simulink model "hw1_model"  (R2024b)
settings: Solver=ode14x  StartTime=0.0  StopTime=44.0  FixedStep=0.001  RelTol=1e-3
undefined symbols (not defined in the file): Cd, Crr, Cxf, Cxr, Cyf, Cyr, F_max_x, F_max_y, Frontal_area, g, J, Jt, lf, lr, m, R, ro, slope
settings Model: Creator=Atakan  LastModifiedBy=Atakan

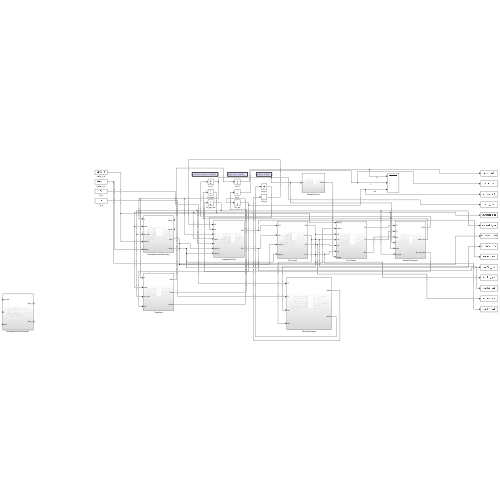
[thumbnail: Simulink's stored preview of the top-level diagram]
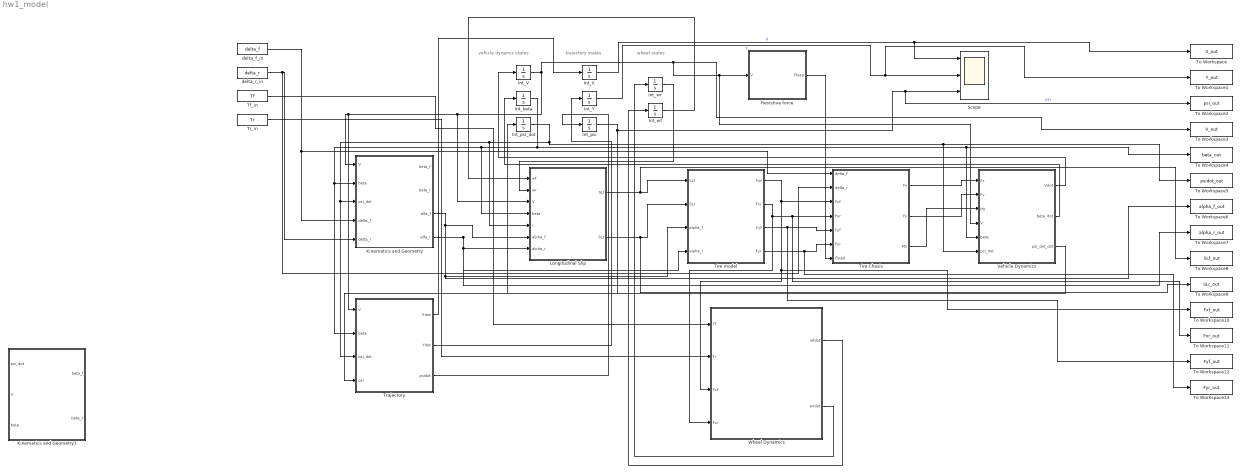
== system hw1_model ==
  note: wheel states
  note: trajectory states
  note: vehicle dynamic states
  Int_V : Integrator
  Int_X : Integrator
  Int_Y : Integrator
  Int_beta : Integrator
  Int_psi : Integrator
  Int_psi_dot : Integrator
  Int_wf : Integrator
  Int_wr : Integrator
  Kinematics and Geometry : Subsystem
  Kinematics and Geometry1 : Subsystem
  Longitudinal Slip : Subsystem
  Resistive force : Subsystem
  Scope : Scope  NumInputPorts=3
  Tf_in : FromWorkspace  VariableName=Tf
  "Tire Chasis " : Subsystem
  Tire model : Subsystem
  To Workspace : ToWorkspace  VariableName=X_out  SaveFormat=Structure With Time  SampleTime=-1
  To Workspace1 : ToWorkspace  VariableName=Y_out  SaveFormat=Structure With Time  SampleTime=-1
  To Workspace10 : ToWorkspace  VariableName=Fxf_out  SaveFormat=Structure With Time  SampleTime=-1
  To Workspace11 : ToWorkspace  VariableName=Fxr_out  SaveFormat=Structure With Time  SampleTime=-1
  To Workspace12 : ToWorkspace  VariableName=Fyf_out  SaveFormat=Structure With Time  SampleTime=-1
  To Workspace13 : ToWorkspace  VariableName=Fyr_out  SaveFormat=Structure With Time  SampleTime=-1
  To Workspace2 : ToWorkspace  VariableName=psi_out  SaveFormat=Structure With Time  SampleTime=-1
  To Workspace3 : ToWorkspace  VariableName=V_out  SaveFormat=Structure With Time  SampleTime=-1
  To Workspace4 : ToWorkspace  VariableName=beta_out  SaveFormat=Structure With Time  SampleTime=-1
  To Workspace5 : ToWorkspace  VariableName=psidot_out  SaveFormat=Structure With Time  SampleTime=-1
  To Workspace6 : ToWorkspace  VariableName=alpha_f_out  SaveFormat=Structure With Time  SampleTime=-1
  To Workspace7 : ToWorkspace  VariableName=alpha_r_out  SaveFormat=Structure With Time  SampleTime=-1
  To Workspace8 : ToWorkspace  VariableName=SLf_out  SaveFormat=Structure With Time  SampleTime=-1
  To Workspace9 : ToWorkspace  VariableName=SLr_out  SaveFormat=Structure With Time  SampleTime=-1
  Tr_in : FromWorkspace  VariableName=Tr
  Trajectory : Subsystem
  Vehicle Dynamics : Subsystem
  Wheel Dynamics : Subsystem
  delta_f_in : FromWorkspace  VariableName=delta_f
  delta_r_in : FromWorkspace  VariableName=delta_r
  wires:
  Int_V/1 -> To Workspace3/1, Vehicle Dynamics/4(V), Resistive force/1(V), Trajectory/1(V), Kinematics and Geometry/1(V), Longitudinal Slip/3(V)
  Int_beta/1 -> To Workspace4/1, Vehicle Dynamics/5(beta), Longitudinal Slip/4(beta), Trajectory/2(beta), Kinematics and Geometry/2(beta)
  Int_psi_dot/1 -> To Workspace5/1, Vehicle Dynamics/6(psi_dot), Longitudinal Slip/5(r), Trajectory/3(psi_dot), Kinematics and Geometry/3(psi_dot)
  delta_f_in/1 -> "Tire Chasis "/1(delta_f), Kinematics and Geometry/4(delta_f)
  delta_r_in/1 -> "Tire Chasis "/2(delta_r), Kinematics and Geometry/5(delta_r)
  Int_wf/1 -> Longitudinal Slip/1(wf)
  Int_wr/1 -> Longitudinal Slip/2(wr)
  Longitudinal Slip/1(SLf) -> To Workspace8/1, Tire model/1(SLf)
  Longitudinal Slip/2(SLr) -> To Workspace9/1, Tire model/2(SLr)
  Kinematics and Geometry/3(alfa_f) -> Longitudinal Slip/6(alpha_f), To Workspace6/1, Tire model/3(alpha_f)
  Kinematics and Geometry/4(alfa_r) -> To Workspace7/1, Longitudinal Slip/7(alpha_r), Tire model/4(alpha_r)
  Tire model/1(Fxf) -> To Workspace10/1, Wheel Dynamics/3(Fxf), "Tire Chasis "/3(Fxf)
  Tire model/2(Fxr) -> Wheel Dynamics/4(Fxr), To Workspace11/1, "Tire Chasis "/4(Fxr)
  Tire model/3(Fyf) -> To Workspace12/1, "Tire Chasis "/5(Fyf)
  Tire model/4(Fyr) -> To Workspace13/1, "Tire Chasis "/6(Fyr)
  Resistive force/1(Fload) -> "Tire Chasis "/7(Fload)
  "Tire Chasis "/1(Fx) -> Vehicle Dynamics/1(Fx)
  "Tire Chasis "/2(Fy) -> Vehicle Dynamics/2(Fy)
  "Tire Chasis "/3(Mz) -> Vehicle Dynamics/3(Mz)
  Vehicle Dynamics/1(Vdot) -> Int_V/1
  Vehicle Dynamics/2(beta_dot) -> Int_beta/1
  Vehicle Dynamics/3(psi_dot_dot) -> Int_psi_dot/1
  Int_psi/1 -> To Workspace2/1, Scope/3, Trajectory/4(psi)  "psi"
  Trajectory/1(Xdot) -> Int_X/1
  Trajectory/2(Ydot) -> Int_Y/1
  Trajectory/3(psidot) -> Int_psi/1
  Tf_in/1 -> Wheel Dynamics/1(Tf)
  Tr_in/1 -> Wheel Dynamics/2(Tr)
  Wheel Dynamics/1(wfdot) -> Int_wf/1
  Wheel Dynamics/2(wrdot) -> Int_wr/1
  Int_X/1 -> To Workspace/1, Scope/1  "X"
  Int_Y/1 -> To Workspace1/1, Scope/2  "Y"

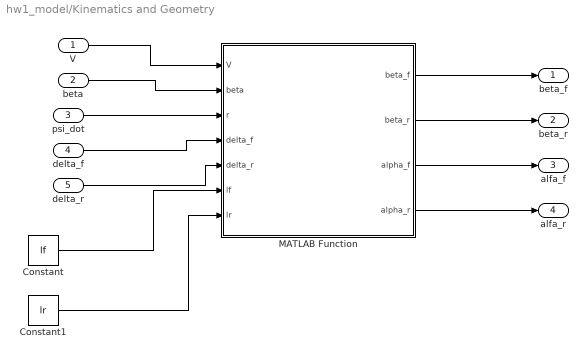
== system hw1_model/Kinematics and Geometry ==
  V : Inport
  beta : Inport  Port=2
  psi_dot : Inport  Port=3
  delta_f : Inport  Port=4
  delta_r : Inport  Port=5
  Constant : Constant  Value=lf
  Constant1 : Constant  Value=lr
  MATLAB Function : MATLAB Function  TreatAsAtomicUnit=on
  beta_f : Outport
  beta_r : Outport  Port=2
  alfa_f : Outport  Port=3
  alfa_r : Outport  Port=4
  wires:
  V/1 -> MATLAB Function/1(V)
  beta/1 -> MATLAB Function/2(beta)
  psi_dot/1 -> MATLAB Function/3(r)
  delta_f/1 -> MATLAB Function/4(delta_f)
  delta_r/1 -> MATLAB Function/5(delta_r)
  Constant/1 -> MATLAB Function/6(lf)
  Constant1/1 -> MATLAB Function/7(lr)
  MATLAB Function/1(beta_f) -> beta_f/1
  MATLAB Function/2(beta_r) -> beta_r/1
  MATLAB Function/3(alpha_f) -> alfa_f/1
  MATLAB Function/4(alpha_r) -> alfa_r/1

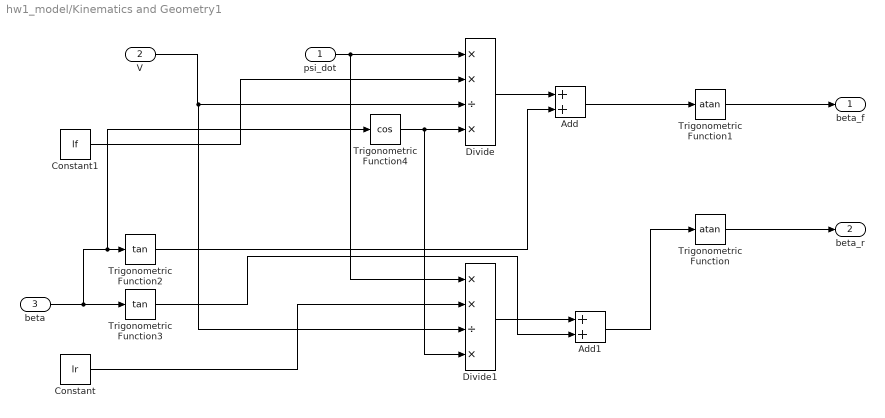
== system hw1_model/Kinematics and Geometry1 ==
  psi_dot : Inport
  V : Inport  Port=2
  beta : Inport  Port=3
  Add : Sum
  Add1 : Sum
  Constant : Constant  Value=lr
  Constant1 : Constant  Value=lf
  Divide : Product  Inputs=**/*
  Divide1 : Product  Inputs=**/*
  Trigonometric Function : Trigonometry  Operator=atan
  Trigonometric Function1 : Trigonometry  Operator=atan
  Trigonometric Function2 : Trigonometry  Operator=tan
  Trigonometric Function3 : Trigonometry  Operator=tan
  Trigonometric Function4 : Trigonometry  Operator=cos
  beta_f : Outport
  beta_r : Outport  Port=2
  wires:
  Trigonometric Function1/1 -> beta_f/1
  Trigonometric Function/1 -> beta_r/1
  beta/1 -> Trigonometric Function4/1, Trigonometric Function2/1, Trigonometric Function3/1
  psi_dot/1 -> Divide1/1, Divide/1
  Constant1/1 -> Divide/2
  V/1 -> Divide1/3, Divide/3
  Trigonometric Function4/1 -> Divide1/4, Divide/4
  Divide/1 -> Add/1
  Trigonometric Function2/1 -> Add/2
  Add/1 -> Trigonometric Function1/1
  Constant/1 -> Divide1/2
  Divide1/1 -> Add1/1
  Trigonometric Function3/1 -> Add1/2
  Add1/1 -> Trigonometric Function/1

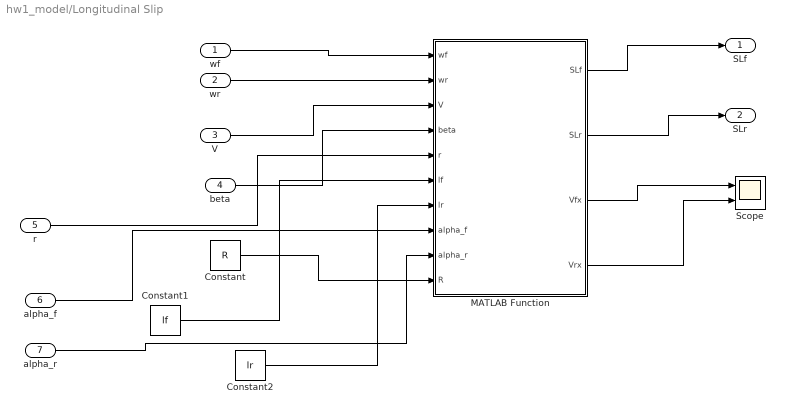
== system hw1_model/Longitudinal Slip ==
  wf : Inport
  wr : Inport  Port=2
  V : Inport  Port=3
  beta : Inport  Port=4
  r : Inport  Port=5
  alpha_f : Inport  Port=6
  alpha_r : Inport  Port=7
  Constant : Constant  Value=R
  Constant1 : Constant  Value=lf
  Constant2 : Constant  Value=lr
  MATLAB Function : MATLAB Function  TreatAsAtomicUnit=on
  Scope : Scope  NumInputPorts=2
  SLf : Outport
  SLr : Outport  Port=2
  wires:
  wf/1 -> MATLAB Function/1(wf)
  wr/1 -> MATLAB Function/2(wr)
  V/1 -> MATLAB Function/3(V)
  beta/1 -> MATLAB Function/4(beta)
  Constant/1 -> MATLAB Function/10(R)
  MATLAB Function/1(SLf) -> SLf/1
  MATLAB Function/2(SLr) -> SLr/1
  MATLAB Function/3(Vfx) -> Scope/1
  MATLAB Function/4(Vrx) -> Scope/2
  Constant1/1 -> MATLAB Function/6(lf)
  Constant2/1 -> MATLAB Function/7(lr)
  r/1 -> MATLAB Function/5(r)
  alpha_f/1 -> MATLAB Function/8(alpha_f)
  alpha_r/1 -> MATLAB Function/9(alpha_r)

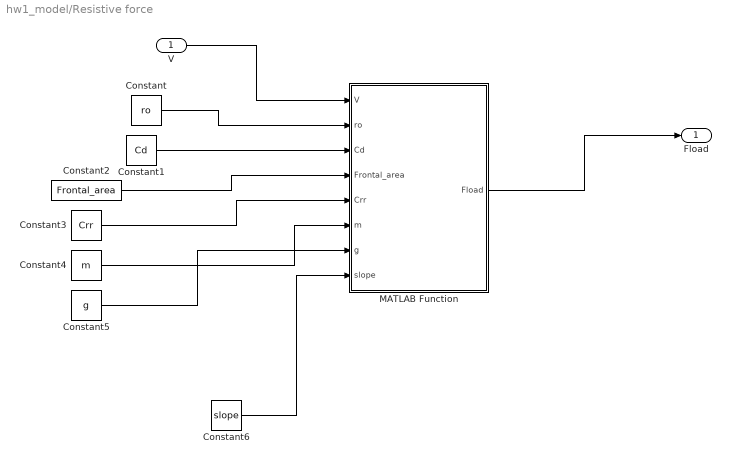
== system hw1_model/Resistive force ==
  V : Inport
  Constant : Constant  Value=ro
  Constant1 : Constant  Value=Cd
  Constant2 : Constant  Value=Frontal_area
  Constant3 : Constant  Value=Crr
  Constant4 : Constant  Value=m
  Constant5 : Constant  Value=g
  Constant6 : Constant  Value=slope
  MATLAB Function : MATLAB Function  TreatAsAtomicUnit=on
  Fload : Outport
  wires:
  V/1 -> MATLAB Function/1(V)
  Constant/1 -> MATLAB Function/2(ro)
  Constant1/1 -> MATLAB Function/3(Cd)
  Constant2/1 -> MATLAB Function/4(Frontal_area)
  Constant3/1 -> MATLAB Function/5(Crr)
  Constant4/1 -> MATLAB Function/6(m)
  Constant5/1 -> MATLAB Function/7(g)
  Constant6/1 -> MATLAB Function/8(slope)
  MATLAB Function/1(Fload) -> Fload/1

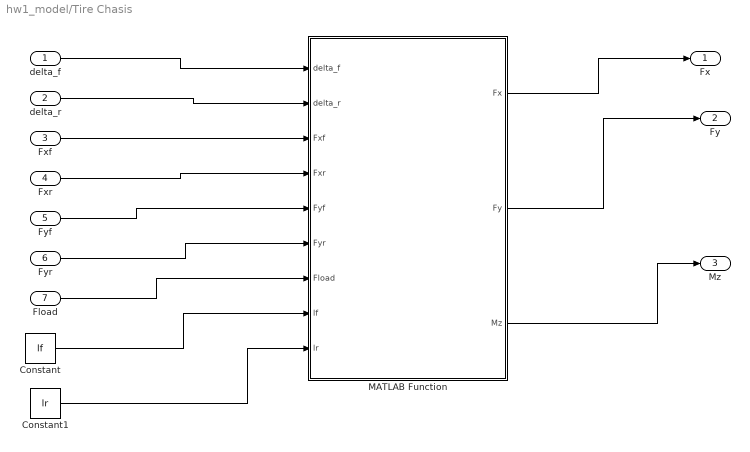
== system hw1_model/Tire Chasis  ==
  delta_f : Inport
  delta_r : Inport  Port=2
  Fxf : Inport  Port=3
  Fxr : Inport  Port=4
  Fyf : Inport  Port=5
  Fyr : Inport  Port=6
  Fload : Inport  Port=7
  Constant : Constant  Value=lf
  Constant1 : Constant  Value=lr
  MATLAB Function : MATLAB Function  TreatAsAtomicUnit=on
  Fx : Outport
  Fy : Outport  Port=2
  Mz : Outport  Port=3
  wires:
  delta_f/1 -> MATLAB Function/1(delta_f)
  delta_r/1 -> MATLAB Function/2(delta_r)
  Fxf/1 -> MATLAB Function/3(Fxf)
  Fxr/1 -> MATLAB Function/4(Fxr)
  Fyf/1 -> MATLAB Function/5(Fyf)
  Fyr/1 -> MATLAB Function/6(Fyr)
  Fload/1 -> MATLAB Function/7(Fload)
  Constant/1 -> MATLAB Function/8(lf)
  Constant1/1 -> MATLAB Function/9(lr)
  MATLAB Function/1(Fx) -> Fx/1
  MATLAB Function/2(Fy) -> Fy/1
  MATLAB Function/3(Mz) -> Mz/1

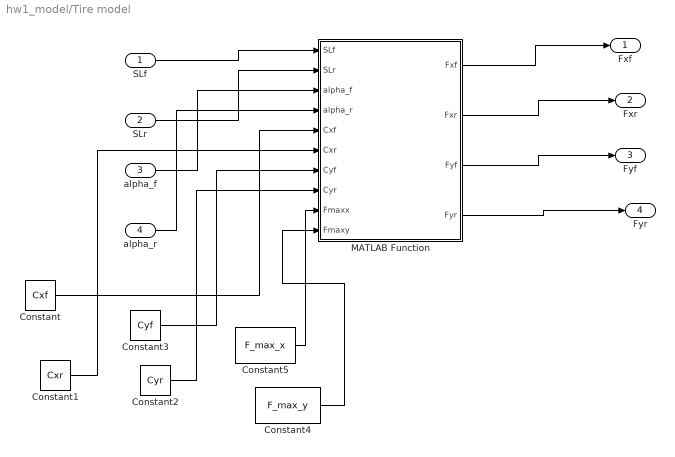
== system hw1_model/Tire model ==
  SLf : Inport
  SLr : Inport  Port=2
  alpha_f : Inport  Port=3
  alpha_r : Inport  Port=4
  Constant : Constant  Value=Cxf
  Constant1 : Constant  Value=Cxr
  Constant2 : Constant  Value=Cyr
  Constant3 : Constant  Value=Cyf
  Constant4 : Constant  Value=F_max_y
  Constant5 : Constant  Value=F_max_x
  MATLAB Function : MATLAB Function  TreatAsAtomicUnit=on
  Fxf : Outport
  Fxr : Outport  Port=2
  Fyf : Outport  Port=3
  Fyr : Outport  Port=4
  wires:
  SLf/1 -> MATLAB Function/1(SLf)
  SLr/1 -> MATLAB Function/2(SLr)
  alpha_f/1 -> MATLAB Function/3(alpha_f)
  alpha_r/1 -> MATLAB Function/4(alpha_r)
  Constant/1 -> MATLAB Function/5(Cxf)
  Constant1/1 -> MATLAB Function/6(Cxr)
  Constant3/1 -> MATLAB Function/7(Cyf)
  Constant2/1 -> MATLAB Function/8(Cyr)
  Constant5/1 -> MATLAB Function/9(Fmaxx)
  Constant4/1 -> MATLAB Function/10(Fmaxy)
  MATLAB Function/1(Fxf) -> Fxf/1
  MATLAB Function/2(Fxr) -> Fxr/1
  MATLAB Function/3(Fyf) -> Fyf/1
  MATLAB Function/4(Fyr) -> Fyr/1

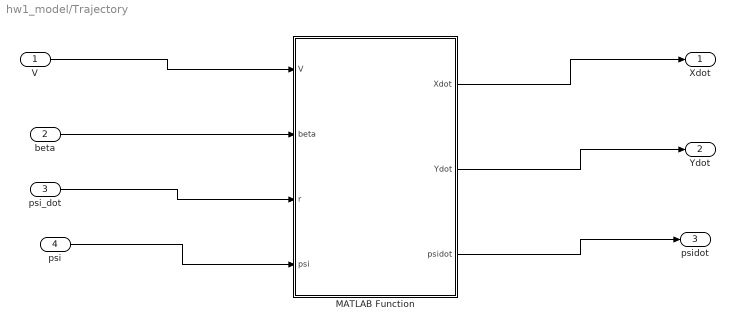
== system hw1_model/Trajectory ==
  V : Inport
  beta : Inport  Port=2
  psi_dot : Inport  Port=3
  psi : Inport  Port=4
  MATLAB Function : MATLAB Function  TreatAsAtomicUnit=on
  Xdot : Outport
  Ydot : Outport  Port=2
  psidot : Outport  Port=3
  wires:
  V/1 -> MATLAB Function/1(V)
  beta/1 -> MATLAB Function/2(beta)
  psi_dot/1 -> MATLAB Function/3(r)
  psi/1 -> MATLAB Function/4(psi)
  MATLAB Function/1(Xdot) -> Xdot/1
  MATLAB Function/2(Ydot) -> Ydot/1
  MATLAB Function/3(psidot) -> psidot/1

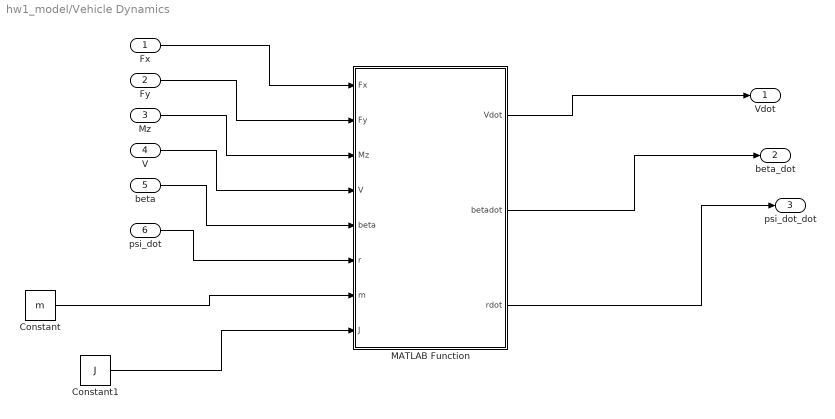
== system hw1_model/Vehicle Dynamics ==
  Fx : Inport
  Fy : Inport  Port=2
  Mz : Inport  Port=3
  V : Inport  Port=4
  beta : Inport  Port=5
  psi_dot : Inport  Port=6
  Constant : Constant  Value=m
  Constant1 : Constant  Value=J
  MATLAB Function : MATLAB Function  TreatAsAtomicUnit=on
  Vdot : Outport
  beta_dot : Outport  Port=2
  psi_dot_dot : Outport  Port=3
  wires:
  Fx/1 -> MATLAB Function/1(Fx)
  Fy/1 -> MATLAB Function/2(Fy)
  Mz/1 -> MATLAB Function/3(Mz)
  V/1 -> MATLAB Function/4(V)
  beta/1 -> MATLAB Function/5(beta)
  psi_dot/1 -> MATLAB Function/6(r)
  Constant/1 -> MATLAB Function/7(m)
  Constant1/1 -> MATLAB Function/8(J)
  MATLAB Function/1(Vdot) -> Vdot/1
  MATLAB Function/2(betadot) -> beta_dot/1
  MATLAB Function/3(rdot) -> psi_dot_dot/1

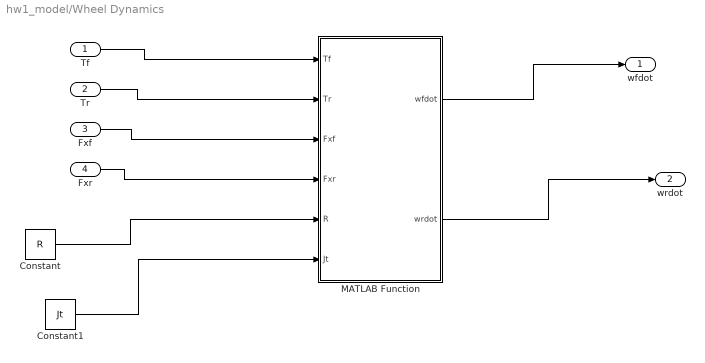
== system hw1_model/Wheel Dynamics ==
  Tf : Inport
  Tr : Inport  Port=2
  Fxf : Inport  Port=3
  Fxr : Inport  Port=4
  Constant : Constant  Value=R
  Constant1 : Constant  Value=Jt
  MATLAB Function : MATLAB Function  TreatAsAtomicUnit=on
  wfdot : Outport
  wrdot : Outport  Port=2
  wires:
  Tf/1 -> MATLAB Function/1(Tf)
  Tr/1 -> MATLAB Function/2(Tr)
  Fxf/1 -> MATLAB Function/3(Fxf)
  Fxr/1 -> MATLAB Function/4(Fxr)
  Constant/1 -> MATLAB Function/5(R)
  Constant1/1 -> MATLAB Function/6(Jt)
  MATLAB Function/1(wfdot) -> wfdot/1
  MATLAB Function/2(wrdot) -> wrdot/1

== matlab function hw1_model/Vehicle Dynamics/MATLAB Function ==
  data: Fx input; Vdot output; Fy input; Mz input; V input; beta input; r input; m input; J input; betadot output; rdot output
function [Vdot,betadot,rdot] = fcn(Fx,Fy,Mz,V,beta,r,m,J)
eps_v = 1e-3;

Vsafe = max(abs(V), eps_v);

Vdot = (Fx*cos(beta) + Fy*sin(beta)) / m;
betadot = (-Fx*sin(beta) + Fy*cos(beta)) / (m*Vsafe) - r;
rdot = Mz / J;

== matlab function hw1_model/Trajectory/MATLAB Function ==
  data: V input; Xdot output; beta input; r input; psi input; Ydot output; psidot output
function [Xdot,Ydot,psidot] = fcn(V,beta,r,psi)
Xdot = V*cos(psi + beta);
Ydot = V*sin(psi + beta);
psidot = r;

== matlab function hw1_model/Wheel Dynamics/MATLAB Function ==
  data: Tf input; wfdot output; Tr input; Fxf input; Fxr input; R input; Jt input; wrdot output
function [wfdot,wrdot] = fcn(Tf,Tr,Fxf,Fxr,R,Jt)
wfdot = (Tf - R*Fxf)/(Jt);
wrdot = (Tr - R*Fxr)/(Jt);

== matlab function hw1_model/Longitudinal Slip/MATLAB Function ==
  data: wf input; wr input; V input; beta input; r input; lf input; lr input; alpha_f input; alpha_r input; SLf output; R input; SLr output; Vfx output; Vrx output
function [SLf,SLr,Vfx,Vrx] = fcn(wf,wr,V,beta,r,lf,lr,alpha_f,alpha_r,R)
eps_s = 1e-3;

% 1. Tekerleklerin ileri bilesen hizlarinin (Vfx, Vrx) dogru hesabi
Vfx = sqrt((V*cos(beta))^2 + (V*sin(beta) + r*lf)^2) * cos(alpha_f);
Vrx = sqrt((V*cos(beta))^2 + (V*sin(beta) - r*lr)^2) * cos(alpha_r);

% 2. Sifira bolme hatalarini engellemek ve dogru paydayi secmek (Hizlanma vs Frenleme)

% On tekerlek icin kayma orani (SLf)
if (wf * R) >= Vfx
    den_f = max(abs(wf * R), eps_s); % Hizlanma
else
    den_f = max(abs(Vfx), eps_s);    % Frenleme
end
SLf = (wf * R - Vfx) / den_f;

% Arka tekerlek icin kayma orani (SLr)
if (wr * R) >= Vrx
    den_r = max(abs(wr * R), eps_s); % Hizlanma
else
    den_r = max(abs(Vrx), eps_s);    % Frenleme
end
SLr = (wr * R - Vrx) / den_r;

== matlab function hw1_model/Kinematics and Geometry/MATLAB Function ==
  data: beta_f output; beta_r output; alpha_f output; alpha_r output; V input; beta input; r input; delta_f input; delta_r input; lf input; lr input
function [beta_f,beta_r,alpha_f,alpha_r] = fcn(V,beta,r,delta_f,delta_r,lf,lr)
eps_v = 1e-3;

den = max(abs(V*cos(beta)), eps_v);

beta_f = atan( tan(beta) + (lf*r)/den );
beta_r = atan( tan(beta) - (lr*r)/den );

alpha_f = delta_f - beta_f;
alpha_r = delta_r - beta_r;

== matlab function hw1_model/Tire model/MATLAB Function ==
  data: SLf input; Fxf output; SLr input; alpha_f input; alpha_r input; Cxf input; Cxr input; Cyf input; Cyr input; Fmaxx input; Fmaxy input; Fxr output; Fyf output; Fyr output
function [Fxf,Fxr,Fyf,Fyr] = fcn(SLf,SLr,alpha_f,alpha_r,Cxf,Cxr,Cyf,Cyr,Fmaxx,Fmaxy)

Fxf = 2 * Cxf * SLf;
Fxr = 2 * Cxr * SLr;
Fyf = 2 * Cyf * alpha_f;
Fyr = 2 * Cyr * alpha_r;

if Fxf > Fmaxx
    Fxf = Fmaxx;
elseif Fxf < -Fmaxx
    Fxf = -Fmaxx;
end

if Fxr > Fmaxx
    Fxr = Fmaxx;
elseif Fxr < -Fmaxx
    Fxr = -Fmaxx;
end

if Fyf > Fmaxy
    Fyf = Fmaxy;
elseif Fyf < -Fmaxy
    Fyf = -Fmaxy;
end

if Fyr > Fmaxy
    Fyr = Fmaxy;
elseif Fyr < -Fmaxy
    Fyr = -Fmaxy;
end

== matlab function hw1_model/Resistive force/MATLAB Function ==
  data: V input; Fload output; ro input; Cd input; Frontal_area input; Crr input; m input; g input; slope input
function Fload = fcn(V,ro,Cd,Frontal_area,Crr,m,g,slope)
% Hiz yonunu yumusak bir sekilde belirlemek icin tanh kullaniyoruz
dir = tanh(50 * V); 

% Kuvvetleri hareket yonune (dir) bagliyoruz
Faero = 0.5 * ro * Cd * Frontal_area * V * abs(V); % V^2 yerine V*abs(V) yonu de korur
Froll = Crr * m * g * dir;
Fgrade = m * g * sin(slope); % Egim hep aynidir

Fload = Faero + Froll + Fgrade;

== matlab function hw1_model/Tire Chasis /MATLAB Function ==
  data: delta_f input; Fx output; delta_r input; Fxf input; Fxr input; Fyf input; Fyr input; Fload input; lf input; lr input; Fy output; Mz output
function [Fx,Fy,Mz] = fcn(delta_f,delta_r,Fxf,Fxr,Fyf,Fyr,Fload,lf,lr)

Fx = -sin(delta_f)*Fyf - sin(delta_r)*Fyr ...
     + cos(delta_f)*Fxf + cos(delta_r)*Fxr ...
     - Fload;

Fy =  cos(delta_f)*Fyf + cos(delta_r)*Fyr ...
     + sin(delta_f)*Fxf + sin(delta_r)*Fxr;

Mz =  lf*cos(delta_f)*Fyf - lr*cos(delta_r)*Fyr ...
     + lf*sin(delta_f)*Fxf - lr*sin(delta_r)*Fxr;
